simulink subsystem "Robot_Control_sub"  (R2026a)
settings: Solver=VariableStepAuto
undefined symbols (not defined in the file): Rebuilt_Hood_Servo_Pos_Max, Rebuilt_Hood_Servo_Pos_Min, TEST_Desired_Hood_Enable_OV, TEST_Desired_Hood_Pos_OV, TEST_Desired_Shooter_FF_DC_OV, TEST_Desired_Shooter_Speed_OV, TEST_Feeder_Motor_DC_OV, TEST_Intake_Arm_Motor_DC_OV, TEST_Intake_Roller_Motor_DC_OV, TEST_Output_Override_Flag, TEST_Transfer_Motor_DC_OV
libraries: Autonomous_lib x1, Disabled_lib x1, Controls_Components_lib x1, Teleop_lib x1, Test_lib x1
(part 1 of 2)
settings Model: Creator=USER  LastModifiedBy=ander

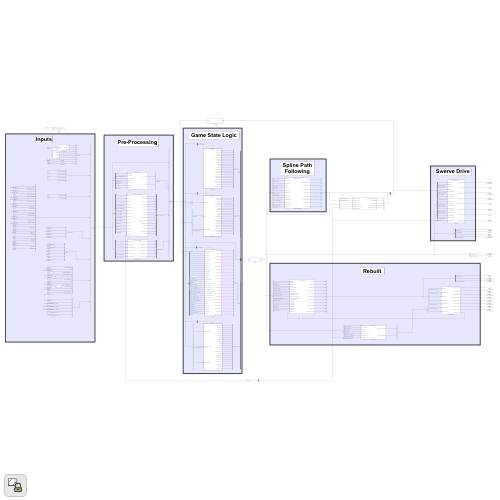
[thumbnail: Simulink's stored preview of the top-level diagram]
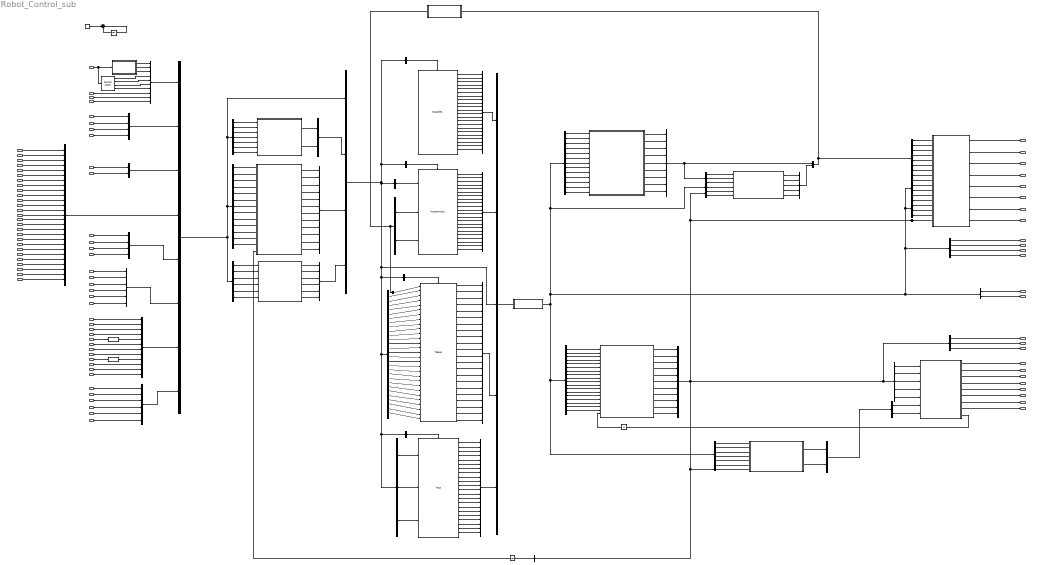
== system Robot_Control_sub ==
  note: Game State Logic
  note: Swerve Drive
  note: Inputs
  note: Pre-Processing
  note: Spline Path
      | Following
  note: Rebuilt
  GameState : Inport
  IsBlueAlliance : Inport  Port=2
  MatchTime : Inport  Port=3
  Xbox_Driver_Stick_Left_X : Inport  Port=4
  Xbox_Driver_Stick_Left_Y : Inport  Port=5
  Xbox_Driver_Bumper_Left : Inport  Port=6
  Xbox_Driver_Stick_Right_X : Inport  Port=7
  Xbox_Driver_Stick_Right_Y : Inport  Port=8
  Xbox_Driver_Bumper_Right : Inport  Port=9
  Xbox_Driver_Trigger_Right : Inport  Port=10
  Xbox_Driver_ButtonY : Inport  Port=11
  Xbox_Driver_ButtonX : Inport  Port=12
  Xbox_Driver_ButtonB : Inport  Port=13
  Xbox_Driver_ButtonA : Inport  Port=14
  Xbox_Driver_Trigger_Left : Inport  Port=15
  Gamepad_Stick_Left_X : Inport  Port=16
  Gamepad_Stick_Left_Y : Inport  Port=17
  Gamepad_Stick_Right_X : Inport  Port=18
  Gamepad_Stick_Right_Y : Inport  Port=19
  Gamepad_B1_A : Inport  Port=20
  Gamepad_B2_B : Inport  Port=21
  Gamepad_B3_X : Inport  Port=22
  Gamepad_B4_Y : Inport  Port=23
  Gamepad_LB : Inport  Port=24
  Gamepad_LT : Inport  Port=25
  Gamepad_RB : Inport  Port=26
  Gamepad_RT : Inport  Port=27
  Gamepad_Back : Inport  Port=28
  Gamepad_Start : Inport  Port=29
  Gamepad_POV : Inport  Port=30
  FL_Drive_Motor_Speed : Inport  Port=31
  FR_Drive_Motor_Speed : Inport  Port=32
  BL_Drive_Motor_Speed : Inport  Port=33
  BR_Drive_Motor_Speed : Inport  Port=34
  Gyro_Angle_Field_rad : Inport  Port=35
  Gyro_Angle_rad : Inport  Port=36
  FL_Steer_Module_Angle : Inport  Port=37
  FR_Steer_Module_Angle : Inport  Port=38
  BL_Steer_Module_Angle : Inport  Port=39
  BR_Steer_Module_Angle : Inport  Port=40
  Odom_Position_X : Inport  Port=41
  Odom_Position_Y : Inport  Port=42
  Odom_Delta_X : Inport  Port=43
  Odom_Delta_Y : Inport  Port=44
  Robot_Velocity_X : Inport  Port=45
  Robot_Velocity_Y : Inport  Port=46
  Vision_Current_Pipeline : Inport  Port=47
  Vision_RobotPoseFieldSpace_X : Inport  Port=48
  Vision_RobotPoseFieldSpace_Y : Inport  Port=49
  Vision_Num_Tags_Detected : Inport  Port=50
  Vision_c1_AprilTag_Valid : Inport  Port=51
  Vision_c1_AprilTag_X_m : Inport  Port=52
  Vision_c1_AprilTag_Y_m : Inport  Port=53
  Vision_c1_AprilTag_Yaw_deg : Inport  Port=54
  Vision_c1_Object_Valid : Inport  Port=55
  Vision_c1_Object_Area_pct : Inport  Port=56
  Vision_c1_Object_Hor_deg : Inport  Port=57
  Vision_c1_Object_Ver_deg : Inport  Port=58
  Measured_Transfer_Speed : Inport  Port=59
  Measured_Shooter_Speed_Left : Inport  Port=60
  Measured_Shooter_Speed_Center : Inport  Port=61
  Measured_Shooter_Speed_Right : Inport  Port=62
  IsBlueInactiveFirst : Inport  Port=63
  Measured_Intake_Arm_Angle : Inport  Port=64
  Measured_Intake_Roller_Speed : Inport  Port=65
  Autonomous : Autonomous_lib/Autonomous  SystemSampleTime=-1  VariantActivationTime=update diagram  EmptyChoice=off  PassThrough=off  PassThroughVariantControl=(default)  EmptyChoiceVariantControl=(default)  AllowFlexibleInterface=on  Latency=0  AutoFrameSizeCalculation=off
  Bus Creator : BusCreator  Inputs=10
  Bus Creator{1..2,4,12} (4 alike) : BusCreator  Inputs=22
  Bus Creator10 : BusCreator  Inputs=11
  Bus Creator11 : BusCreator  Inputs=8
  Bus Creator13 : BusCreator  Inputs=9
  Bus Creator{14,16,19..20} (4 alike) : BusCreator  Inputs=2
  Bus Creator15 : BusCreator  Inputs=5
  Bus Creator17 : BusCreator  Inputs=4
  Bus Creator18 : BusCreator  Inputs=12
  Bus Creator21 : BusCreator  Inputs=6
  Bus Creator24 : BusCreator  Inputs=12
  Bus Creator3 : BusCreator  Inputs=5
  Bus Creator5 : BusCreator  Inputs=27
  Bus Creator6 : BusCreator  Inputs=6
  Bus Creator7 : BusCreator  Inputs=4
  Bus Creator8 : BusCreator  Inputs=4
  Bus Creator9 : BusCreator  Inputs=6
  Bus Selector : BusSelector  OutputSignals=Desired_Gyro_Override.Steering_Abs_Cmd,SPF.Steering_Rel_Cmd_SPF,SPF.Translation_Speed_SPF,SPF.Translation_Angle_SPF,SPF.Is_Absolute_Translation_SPF,Desired_Gyro_Override.Is_Absolute_Steering,Desired_Gyro_Override.Gyro_Angle_Steering_rad,Desired_Gyro_Override.Gyro_Angle_Translation_rad
  Bus Selector1 : BusSelector  OutputSignals=PreProcessing.Inputs.Game_States.GameState,PreProcessing.Inputs.Game_States.IsBlueAlliance,PreProcessing.Inputs.Game_States.IsBlueInactiveFirst,PreProcessing.Inputs.Game_States.MatchTime,Button_Spinup_Enable,Button_Shoot_Enable,PreProcessing.Inputs.Human_Inputs_Raw.Gamepad_RT,PreProcessing.Inputs.Rebuilt_Specific.Measured_Transfer_Speed,PreProcessing.Inputs.Rebuilt_Specific.Measured_Shooter_Speed_Left,PreProcessing.Inputs.Rebuilt_Specific.Measured_Shooter_Speed_Center,PreProcessing.Inputs.Rebuilt_Specific.Measured_Shooter_Speed_Right,PreProcessing.Inputs.Gyro.Gyro_Angle_Field_rad,PreProcessing.Kalman_Filter.KF_Position_X,PreProcessing.Kalman_Filter.KF_Position_Y,PreProcessing.Inputs.Odometry.Robot_Velocity_X,PreProcessing.Inputs.Odometry.Robot_Velocity_Y,PreProcessing.Inputs.Human_Inputs_Raw.Gamepad_B2_B,PreProcessing.Inputs.Human_Inputs_Raw.Gamepad_Start
  Bus Selector10 : BusSelector  OutputSignals=Is_Absolute_Steering_SPF,Steering_Abs_Cmd_SPF,Gyro_Angle_SPF
  Bus Selector11 : BusSelector  OutputSignals=PreProcessing.Inputs.Gyro.Gyro_Angle_Field_rad
  Bus Selector12 : BusSelector  OutputSignals=Rebuilt_Intake_Arm_Motor_DC,RB_Intake_Roller_Motor_PID_DC
  Bus Selector13 : BusSelector  OutputSignals=Human_Inputs_Raw.Xbox_Driver_Stick_Left_X,Human_Inputs_Raw.Xbox_Driver_Stick_Left_Y,Human_Inputs_Raw.Xbox_Driver_Stick_Right_X,Human_Inputs_Raw.Xbox_Driver_Stick_Right_Y,Human_Inputs_Raw.Xbox_Driver_Trigger_Right,Human_Inputs_Raw.Xbox_Driver_ButtonY,Human_Inputs_Raw.Xbox_Driver_ButtonX,Human_Inputs_Raw.Xbox_Driver_ButtonB,Human_Inputs_Raw.Xbox_Driver_ButtonA,Human_Inputs_Raw.Gamepad_B3_X,Human_Inputs_Raw.Gamepad_B4_Y,Human_Inputs_Raw.Gamepad_B2_B,Gyro.Gyro_Angle_rad
  Bus Selector14 : BusSelector  OutputSignals=Intake_Arm_Move_In,Intake_Arm_Move_Out,Intake_Arm_Cycle,Intake_Roller_On,PreProcessing.Inputs.Rebuilt_Specific.Measured_Intake_Arm_Angle,PreProcessing.Inputs.Rebuilt_Specific.Measured_Intake_Roller_Speed
  Bus Selector15 : BusSelector  OutputSignals=Spline_Index,Robot_Reached_Destination
  Bus Selector16 : BusSelector  OutputSignals=Human_Inputs_Processed.Button_Enable_Wheels,Human_Inputs_Processed.Button_Reset_Wheel_Offsets,Human_Inputs_Processed.Button_Disable_Wheels
  Bus Selector17 : BusSelector  OutputSignals=Field_Angle_Override_Enable
  Bus Selector18 : BusSelector  OutputSignals=Enable_Wheels,Reset_Wheel_Offsets,Disable_Wheels,Swerve_Motors_Disabled
  Bus Selector19 : BusSelector  OutputSignals=Desired_Pipeline,Auto_Initial_Gyro_Angle
  Bus Selector2 : BusSelector  OutputSignals=Inputs.Game_States.Game_State_Teleop
  Bus Selector20 : BusSelector  OutputSignals=Vision_Estimates.Vision_c1_AprilTag_X_m,Vision_Estimates.Vision_c1_AprilTag_Y_m,Vision_Estimates.Vision_c1_AprilTag_Yaw_deg,Vision_Estimates.Vision_c1_Object_Area_pct,Vision_Estimates.Vision_c1_Object_Hor_deg,Vision_Estimates.Vision_c1_Object_Ver_deg
  Bus Selector22 : BusSelector  OutputSignals=Shooter_Active
  Bus Selector23 : BusSelector  OutputSignals=Aim_Active
  Bus Selector24 : BusSelector  OutputSignals=Shooter_Motor_Gain_Kp,Shooter_Motor_Gain_Ki,Shooter_Motor_Gain_Change
  Bus Selector25 : BusSelector  OutputSignals=RB_Transfer_Motor_PID_DC
  Bus Selector3 : BusSelector  OutputSignals=Vision_Estimates.Vision_RobotPoseFieldSpace_X,Vision_Estimates.Vision_RobotPoseFieldSpace_Y,Vision_Estimates.Vision_Num_Tags_Detected,Odometry.Odom_Position_X,Odometry.Odom_Position_Y,Odometry.Odom_Delta_X,Odometry.Odom_Delta_Y
  Bus Selector4 : BusSelector  OutputSignals=Inputs.Game_States.Game_State_Auto
  Bus Selector41 : BusSelector  OutputSignals=Human_Inputs_Processed.Drive_Joystick_X,Human_Inputs_Processed.Drive_Joystick_Y,Human_Inputs_Processed.Steer_Joystick_X,Human_Inputs_Processed.Steer_Joystick_Y,Human_Inputs_Processed.Drive_Speed_Boost,Human_Inputs_Processed.Face_Toward_Driver,Human_Inputs_Processed.Face_Right_Driver,Human_Inputs_Processed.Face_Left_Driver,Human_Inputs_Processed.Face_Away_Driver,Inputs.Gyro.Gyro_Angle_rad,Inputs.Game_States.Prev_Active_GameState,Inputs.Game_States.IsBlueAlliance,Inputs.Vision_Estimates.Vision_Current_Pipeline,Inputs.Vision_Estimates.Vision_c1_AprilTag_Valid,Vision_Corrected.Vision_c1_AprilTag_Corr_X_inch,Vision_Corrected.Vision_c1_AprilTag_Corr_Y_inch,Vision_Corrected.Vision_c1_AprilTag_Corr_Yaw_deg,Inputs.Vision_Estimates.Vision_c1_Object_Valid,Vision_Corrected.Vision_c1_Object_Corr_X_inch,Vision_Corrected.Vision_c1_Object_Corr_Y_inch,Vision_Corrected.Vision_c1_Object_Corr_Yaw_deg,Inputs.Human_Inputs_Raw.Gamepad_LB,Inputs.Human_Inputs_Raw.Gamepad_RB,Inputs.Human_Inputs_Raw.Gamepad_B1_A,Inputs.Human_Inputs_Raw.Gamepad_B4_Y,Inputs.Human_Inputs_Raw.Gamepad_B3_X,Inputs.Human_Inputs_Raw.Xbox_Driver_Trigger_Left,Inputs.Human_Inputs_Raw.Gamepad_LT
  Bus Selector5 : BusSelector  OutputSignals=Aim_Active,RB_Desired_Shoot_Gyro_Ang
  Bus Selector50 : BusSelector  OutputSignals=PreProcessing.Inputs.Drive_Motor_Speeds.FL_Drive_Motor_Speed,PreProcessing.Inputs.Drive_Motor_Speeds.FR_Drive_Motor_Speed,PreProcessing.Inputs.Drive_Motor_Speeds.BL_Drive_Motor_Speed,PreProcessing.Inputs.Drive_Motor_Speeds.BR_Drive_Motor_Speed
  Bus Selector52 : BusSelector  OutputSignals=PreProcessing.Inputs.Steer_Module_Angles.FL_Steer_Module_Angle,PreProcessing.Inputs.Steer_Module_Angles.FR_Steer_Module_Angle,PreProcessing.Inputs.Steer_Module_Angles.BL_Steer_Module_Angle,PreProcessing.Inputs.Steer_Module_Angles.BR_Steer_Module_Angle
  Bus Selector59 : BusSelector  OutputSignals=Inputs.Game_States.IsBlueAlliance
  Bus Selector6 : BusSelector  OutputSignals=Inputs.Game_States.Game_State_Disabled
  Bus Selector7 : BusSelector  OutputSignals=RB_Transfer_Motor_PID_DC,RB_Feeder_Motor_PID_DC,RB_Desired_Hood_Pos_Shoot,RB_Desired_Shooter_Speed,Desired_Shooter_FF_DC
  Bus Selector8 : BusSelector  OutputSignals=Inputs.Game_States.Game_State_Test
  Bus Selector9 : BusSelector  OutputSignals=Spline_Enable,Spline_Ref_Poses,Spline_Num_Poses,PreProcessing.Kalman_Filter.KF_Position_X,PreProcessing.Kalman_Filter.KF_Position_Y,Steering_Abs_Cmd,Steering_Rel_Cmd,Translation_Speed,Translation_Angle,Is_Absolute_Translation,Is_Absolute_Steering,PreProcessing.Inputs.Gyro.Gyro_Angle_Field_rad,PreProcessing.Inputs.Gyro.Gyro_Angle_rad
  Constant2 : Constant
  Data Type Conversion : DataTypeConversion  OutDataTypeStr=boolean  SaturateOnIntegerOverflow=off  RndMeth=Floor
  Data Type Conversion1 : DataTypeConversion  OutDataTypeStr=boolean  SaturateOnIntegerOverflow=off  RndMeth=Floor
  Desired Gyro Override for Shooting : Subsystem
  Disabled : Disabled_lib/Disabled  SystemSampleTime=-1  VariantActivationTime=update diagram  EmptyChoice=off  PassThrough=off  PassThroughVariantControl=(default)  EmptyChoiceVariantControl=(default)  AllowFlexibleInterface=on  Latency=0  AutoFrameSizeCalculation=off
  Human_Input_Pre_Processing : Subsystem  ReferencedSubsystem=Human_Input_Pre_Processing_sub
  Intake Controls : Subsystem  ReferencedSubsystem=Intake_Controls_sub
  Internal Feedback : Subsystem
  Kalman_Filter : Subsystem  ReferencedSubsystem=Kalman_Filter_sub
  Merge : Subsystem
  Output Overrides : Subsystem
  Previous GameState : Subsystem
  Shooter Controls : Subsystem  ReferencedSubsystem=Shooter_Controls_sub
  Spline_Path_Following : Subsystem  ReferencedSubsystem=Spline_Path_Following_sub
  Sum : Sum  Inputs=|++
  Swerve_Drive : Subsystem  ReferencedSubsystem=Swerve_Drive_sub
  Switch Case : SwitchCase  CaseConditions={0,1,2}
  Teleop : Teleop_lib/Teleop  SystemSampleTime=-1  VariantActivationTime=update diagram  EmptyChoice=off  PassThrough=off  PassThroughVariantControl=(default)  EmptyChoiceVariantControl=(default)  AllowFlexibleInterface=on  Latency=0  AutoFrameSizeCalculation=off
  Test : Test_lib/Test  SystemSampleTime=-1  VariantActivationTime=update diagram  EmptyChoice=off  PassThrough=off  PassThroughVariantControl=(default)  EmptyChoiceVariantControl=(default)  AllowFlexibleInterface=on  Latency=0  AutoFrameSizeCalculation=off
  Unit Delay : UnitDelay  SampleTime=-1
  Unit Delay1 : UnitDelay  SampleTime=-1
  Unit Delay2 : UnitDelay  SampleTime=-1
  Vision_Corrections : Subsystem  ReferencedSubsystem=Vision_Corrections_sub
  FL_Steering_Motor_DC : Outport
  FL_Drive_Motor_DC : Outport  Port=2
  FR_Steering_Motor_DC : Outport  Port=3
  FR_Drive_Motor_DC : Outport  Port=4
  BL_Steering_Motor_DC : Outport  Port=5
  BL_Drive_Motor_DC : Outport  Port=6
  BR_Steering_Motor_DC : Outport  Port=7
  BR_Drive_Motor_DC : Outport  Port=8
  Enable_Wheels : Outport  Port=9
  Reset_Wheel_Offsets : Outport  Port=10
  Disable_Wheels : Outport  Port=11
  Swerve_Motors_Disabled : Outport  Port=12
  Vision_Desired_Pipeline : Outport  Port=13
  Transfer_Motor_DC : Outport  Port=14
  Feeder_Motor_DC : Outport  Port=15
  Desired_Shooter_Speed : Outport  Port=16
  Desired_Shooter_FF_DC : Outport  Port=17
  Desired_Hood_Enable : Outport  Port=18
  Desired_Hood_Pos : Outport  Port=19
  Intake_Arm_Motor_DC : Outport  Port=20
  Intake_Roller_Motor_DC : Outport  Port=21
  Auto_Initial_Gyro_Angle : Outport  Port=22
  Shooter_Motor_Gain_Kp : Outport  Port=23
  Shooter_Motor_Gain_Ki : Outport  Port=24
  Shooter_Motor_Gain_Change : Outport  Port=25
  wires:
  Bus Creator4/1 -> Bus Creator3/1  "Disabled"
  Bus Creator1/1 -> Bus Creator3/2  "Autonomous"
  Bus Creator2/1 -> Bus Creator3/4  "Teleop"
  Switch Case/1 -> Bus Creator/4  "Game_State_Disabled"
  Switch Case/2 -> Bus Creator/5  "Game_State_Auto"
  Switch Case/3 -> Bus Creator/6  "Game_State_Teleop"
  GameState/1 -> Previous GameState/1(GameState_in), Switch Case/1  "GameState"
  Bus Creator12/1 -> Bus Creator3/5  "Test"
  Switch Case/4 -> Bus Creator/7  "Game_State_Test"
  FL_Drive_Motor_Speed/1 -> Bus Creator7/1  "FL_Drive_Motor_Speed"
  FR_Drive_Motor_Speed/1 -> Bus Creator7/2  "FR_Drive_Motor_Speed"
  BL_Drive_Motor_Speed/1 -> Bus Creator7/3  "BL_Drive_Motor_Speed"
  BR_Drive_Motor_Speed/1 -> Bus Creator7/4  "BR_Drive_Motor_Speed"
  Bus Creator/1 -> Bus Creator11/1  "Game_States"
  Bus Selector2/1 -> Teleop/Action  "<Game_State_Teleop>"
  Bus Selector4/1 -> Autonomous/Action  "<Game_State_Auto>"
  Bus Selector6/1 -> Disabled/Action  "<Game_State_Disabled>"
  Bus Selector8/1 -> Test/Action  "<Game_State_Test>"
  Bus Selector50/4 -> Swerve_Drive/12  "<BR_Drive_Motor_Speed>"
  Bus Selector50/3 -> Swerve_Drive/11  "<BL_Drive_Motor_Speed>"
  Bus Selector50/2 -> Swerve_Drive/10  "<FR_Drive_Motor_Speed>"
  Bus Selector50/1 -> Swerve_Drive/9  "<FL_Drive_Motor_Speed>"
  Swerve_Drive/1 -> FL_Steering_Motor_DC/1
  Swerve_Drive/2 -> FL_Drive_Motor_DC/1
  Swerve_Drive/3 -> FR_Steering_Motor_DC/1
  Swerve_Drive/4 -> FR_Drive_Motor_DC/1
  Swerve_Drive/5 -> BL_Steering_Motor_DC/1
  Swerve_Drive/6 -> BL_Drive_Motor_DC/1
  Swerve_Drive/7 -> BR_Steering_Motor_DC/1
  Swerve_Drive/8 -> BR_Drive_Motor_DC/1
  Xbox_Driver_Trigger_Right/1 -> Bus Creator5/8  "Xbox_Driver_Trigger_Right"
  Gyro_Angle_Field_rad/1 -> Bus Creator14/1  "Gyro_Angle_Field_rad"
  Gyro_Angle_rad/1 -> Bus Creator14/2  "Gyro_Angle_rad"
  Bus Creator11/1 -> Bus Selector20/1, Bus Selector13/1, Bus Selector3/1, Bus Creator17/1  "Inputs"
  Bus Selector52/1 -> Swerve_Drive/13  "<FL_Steer_Module_Angle>"
  Bus Selector52/2 -> Swerve_Drive/14  "<FR_Steer_Module_Angle>"
  Bus Selector52/3 -> Swerve_Drive/15  "<BL_Steer_Module_Angle>"
  Bus Selector52/4 -> Swerve_Drive/16  "<BR_Steer_Module_Angle>"
  Merge/1(Bus_Out) -> Bus Selector11/1, Bus Selector9/1, Bus Selector19/1, Bus Selector18/1, Bus Selector52/1, Bus Selector50/1, Bus Selector1/1, Bus Selector14/1
  Bus Creator3/1 -> Merge/1(Bus_In)
  Bus Selector9/1 -> Spline_Path_Following/1  "<Spline_Enable>"
  Bus Selector9/2 -> Spline_Path_Following/2  "<Spline_Ref_Poses>"
  Bus Selector9/3 -> Spline_Path_Following/3  "<Spline_Num_Poses>"
  Bus Selector9/7 -> Spline_Path_Following/7  "<Steering_Rel_Cmd>"
  Bus Selector9/8 -> Spline_Path_Following/8  "<Translation_Speed>"
  Bus Selector9/9 -> Spline_Path_Following/9  "<Translation_Angle>"
  Bus Selector9/10 -> Spline_Path_Following/10  "<Is_Absolute_Translation>"
  Bus Selector9/11 -> Spline_Path_Following/11  "<Is_Absolute_Steering>"
  Spline_Path_Following/3 -> Bus Creator13/3
  Spline_Path_Following/4 -> Bus Creator13/4
  Spline_Path_Following/5 -> Bus Creator13/5
  Spline_Path_Following/6 -> Bus Creator13/6
  Spline_Path_Following/7 -> Bus Creator13/7
  Spline_Path_Following/8 -> Bus Creator13/8
  Bus Creator13/1 -> Bus Creator16/1, Bus Selector10/1  "SPF"
  Bus Selector/5 -> Swerve_Drive/5  "<Is_Absolute_Translation_SPF>"
  Bus Selector/4 -> Swerve_Drive/4  "<Translation_Angle_SPF>"
  Bus Selector/6 -> Swerve_Drive/6  "<Is_Absolute_Steering>"
  Bus Selector/3 -> Swerve_Drive/3  "<Translation_Speed_SPF>"
  Bus Selector/2 -> Swerve_Drive/2  "<Steering_Rel_Cmd_SPF>"
  Bus Selector/1 -> Swerve_Drive/1  "<Steering_Abs_Cmd>"
  Spline_Path_Following/2 -> Bus Creator13/2
  Vision_RobotPoseFieldSpace_X/1 -> Bus Creator18/2  "Vision_RobotPoseFieldSpace_X"
  Vision_RobotPoseFieldSpace_Y/1 -> Bus Creator18/3  "Vision_RobotPoseFieldSpace_Y"
  Vision_Num_Tags_Detected/1 -> Bus Creator18/4  "Vision_Num_Tags_Detected"
  Bus Selector3/3 -> Kalman_Filter/3  "<Vision_Num_Tags_Detected>"
  Bus Selector3/2 -> Kalman_Filter/2  "<Vision_RobotPoseFieldSpace_Y>"
  Bus Selector3/1 -> Kalman_Filter/1  "<Vision_RobotPoseFieldSpace_X>"
  Kalman_Filter/1 -> Bus Creator19/1
  Kalman_Filter/2 -> Bus Creator19/2
  Bus Selector9/4 -> Spline_Path_Following/4  "<KF_Position_X>"
  Bus Selector9/5 -> Spline_Path_Following/5  "<KF_Position_Y>"
  Bus Creator19/1 -> Bus Creator17/2  "Kalman_Filter"
  Xbox_Driver_ButtonB/1 -> Bus Creator5/11  "Xbox_Driver_ButtonB"
  Xbox_Driver_ButtonX/1 -> Bus Creator5/10  "Xbox_Driver_ButtonX"
  Xbox_Driver_ButtonY/1 -> Bus Creator5/9  "Xbox_Driver_ButtonY"
  Bus Selector13/3 -> Human_Input_Pre_Processing/3  "<Xbox_Driver_Stick_Right_X>"
  Bus Selector13/4 -> Human_Input_Pre_Processing/4  "<Xbox_Driver_Stick_Right_Y>"
  Bus Selector13/1 -> Human_Input_Pre_Processing/1  "<Xbox_Driver_Stick_Left_X>"
  Bus Selector13/2 -> Human_Input_Pre_Processing/2  "<Xbox_Driver_Stick_Left_Y>"
  Bus Selector13/5 -> Human_Input_Pre_Processing/5  "<Xbox_Driver_Trigger_Right>"
  Xbox_Driver_Stick_Left_Y/1 -> Bus Creator5/2  "Xbox_Driver_Stick_Left_Y"
  Xbox_Driver_Stick_Left_X/1 -> Bus Creator5/1  "Xbox_Driver_Stick_Left_X"
  Xbox_Driver_Bumper_Left/1 -> Bus Creator5/5  "Xbox_Driver_Bumper_Left"
  Xbox_Driver_Stick_Right_X/1 -> Bus Creator5/3  "Xbox_Driver_Stick_Right_X"
  Xbox_Driver_Stick_Right_Y/1 -> Bus Creator5/4  "Xbox_Driver_Stick_Right_Y"
  Xbox_Driver_Bumper_Right/1 -> Bus Creator5/6  "Xbox_Driver_Bumper_Right"
  Bus Creator24/1 -> Bus Creator17/3  "Human_Inputs_Processed"
  Bus Creator17/1 -> Bus Selector4/1, Bus Selector6/1, Bus Creator3/3, Bus Selector2/1, Bus Selector41/1, Bus Selector8/1, Bus Selector16/1, Bus Selector59/1  "PreProcessing"
  Bus Creator18/1 -> Bus Creator11/7  "Vision_Estimates"
  Vision_c1_AprilTag_X_m/1 -> Bus Creator18/6  "Vision_c1_AprilTag_X_m"
  Vision_c1_AprilTag_Y_m/1 -> Bus Creator18/7  "Vision_c1_AprilTag_Y_m"
  Previous GameState/1(GameState) -> Bus Creator/1
  Previous GameState/3(Prev_Active_GameState) -> Bus Creator/3
  IsBlueAlliance/1 -> Bus Creator/8  "IsBlueAlliance"
  Bus Selector9/12 -> Spline_Path_Following/12  "<Gyro_Angle_Field_rad>"
  Bus Selector9/13 -> Spline_Path_Following/13  "<Gyro_Angle_rad>"
  Spline_Path_Following/9 -> Bus Creator13/9
  Bus Selector59/1 -> Autonomous/1  "<IsBlueAlliance>"
  Bus Selector18/2 -> Reset_Wheel_Offsets/1  "<Reset_Wheel_Offsets>"
  Bus Selector18/3 -> Disable_Wheels/1  "<Disable_Wheels>"
  Bus Selector18/4 -> Swerve_Motors_Disabled/1  "<Swerve_Motors_Disabled>"
  Bus Selector18/1 -> Enable_Wheels/1  "<Enable_Wheels>"
  Bus Selector16/1 -> Test/1  "<Button_Enable_Wheels>"
  Bus Selector16/2 -> Test/2  "<Button_Reset_Wheel_Offsets>"
  Bus Selector16/3 -> Test/3  "<Button_Disable_Wheels>"
  Xbox_Driver_ButtonA/1 -> Bus Creator5/12  "Xbox_Driver_ButtonA"
  Xbox_Driver_Trigger_Left/1 -> Bus Creator5/7  "Xbox_Driver_Trigger_Left"
  Gamepad_Stick_Left_X/1 -> Bus Creator5/13  "Gamepad_Stick_Left_X"
  Gamepad_Stick_Left_Y/1 -> Bus Creator5/14  "Gamepad_Stick_Left_Y"
  Gamepad_Stick_Right_X/1 -> Bus Creator5/15  "Gamepad_Stick_Right_X"
  Gamepad_Stick_Right_Y/1 -> Bus Creator5/16  "Gamepad_Stick_Right_Y"
  Gamepad_B1_A/1 -> Bus Creator5/17  "Gamepad_B1_A"
  Gamepad_B2_B/1 -> Bus Creator5/18  "Gamepad_B2_B"
  Gamepad_B3_X/1 -> Bus Creator5/19  "Gamepad_B3_X"
  Gamepad_B4_Y/1 -> Bus Creator5/20  "Gamepad_B4_Y"
  Gamepad_LB/1 -> Bus Creator5/21  "Gamepad_LB"
  Gamepad_LT/1 -> Bus Creator5/22  "Gamepad_LT"
  Gamepad_RB/1 -> Bus Creator5/23  "Gamepad_RB"
  Gamepad_RT/1 -> Bus Creator5/24  "Gamepad_RT"
  Gamepad_Back/1 -> Bus Creator5/25  "Gamepad_Back"
  Gamepad_Start/1 -> Bus Creator5/26  "Gamepad_Start"
  Bus Creator5/1 -> Bus Creator11/4  "Human_Inputs_Raw"
  Gamepad_POV/1 -> Bus Creator5/27  "Gamepad_POV"
  Vision_Corrections/1 -> Bus Creator21/1
  Vision_Corrections/2 -> Bus Creator21/2
  Vision_Corrections/3 -> Bus Creator21/3
  Bus Creator21/1 -> Bus Creator17/4  "Vision_Corrected"
  Previous GameState/2(Prev_GameState) -> Bus Creator/2
  MatchTime/1 -> Bus Creator/9  "MatchTime"
  Odom_Position_X/1 -> Bus Creator9/1  "Odom_Position_X"
  Odom_Position_Y/1 -> Bus Creator9/2  "Odom_Position_Y"
  Odom_Delta_X/1 -> Bus Creator9/3  "Odom_Delta_X"
  Odom_Delta_Y/1 -> Bus Creator9/4  "Odom_Delta_Y"
  Bus Creator9/1 -> Bus Creator11/6  "Odometry"
  BR_Steer_Module_Angle/1 -> Bus Creator8/4  "BR_Steer_Module_Angle"
  BL_Steer_Module_Angle/1 -> Bus Creator8/3  "BL_Steer_Module_Angle"
  FR_Steer_Module_Angle/1 -> Bus Creator8/2  "FR_Steer_Module_Angle"
  FL_Steer_Module_Angle/1 -> Bus Creator8/1  "FL_Steer_Module_Angle"
  Bus Creator7/1 -> Bus Creator11/2  "Drive_Motor_Speeds"
  Bus Creator14/1 -> Bus Creator11/3  "Gyro"
  Constant2/1 -> Sum/1
  Unit Delay1/1 -> Sum/2
  Sum/1 -> Unit Delay1/1  "loop_counter_robot_control"
  Vision_c1_AprilTag_Yaw_deg/1 -> Bus Creator18/8  "Vision_c1_AprilTag_Yaw_deg"
  Teleop/1 -> Bus Creator2/1
  Teleop/2 -> Bus Creator2/2
  Teleop/3 -> Bus Creator2/3
  Teleop/4 -> Bus Creator2/4
  Teleop/5 -> Bus Creator2/5
  Teleop/6 -> Bus Creator2/6
  Teleop/7 -> Bus Creator2/7
  Test/1 -> Bus Creator12/1
  Test/2 -> Bus Creator12/2
  Test/3 -> Bus Creator12/3
  Test/4 -> Bus Creator12/4
  Test/5 -> Bus Creator12/5
  Test/6 -> Bus Creator12/6
  Test/7 -> Bus Creator12/7
  Test/8 -> Bus Creator12/8
  Test/9 -> Bus Creator12/9
  Test/10 -> Bus Creator12/10
  Test/11 -> Bus Creator12/11
  Test/12 -> Bus Creator12/12
  Test/13 -> Bus Creator12/13
  Test/14 -> Bus Creator12/14
  Disabled/1 -> Bus Creator4/1
  Disabled/2 -> Bus Creator4/2
  Disabled/3 -> Bus Creator4/3
  Disabled/4 -> Bus Creator4/4
  Disabled/5 -> Bus Creator4/5
  Disabled/6 -> Bus Creator4/6
  Disabled/7 -> Bus Creator4/7
  Disabled/8 -> Bus Creator4/8
  Disabled/9 -> Bus Creator4/9
  Disabled/10 -> Bus Creator4/10
  Disabled/11 -> Bus Creator4/11
  Disabled/12 -> Bus Creator4/12
  Disabled/13 -> Bus Creator4/13
  Disabled/14 -> Bus Creator4/14
  Autonomous/1 -> Bus Creator1/1
  Autonomous/2 -> Bus Creator1/2
  Autonomous/3 -> Bus Creator1/3
  Autonomous/4 -> Bus Creator1/4
  Autonomous/5 -> Bus Creator1/5
  Autonomous/6 -> Bus Creator1/6
  Autonomous/7 -> Bus Creator1/7
  Autonomous/8 -> Bus Creator1/8
  Autonomous/9 -> Bus Creator1/9
  Autonomous/10 -> Bus Creator1/10
  Autonomous/11 -> Bus Creator1/11
  Autonomous/12 -> Bus Creator1/12
  Autonomous/13 -> Bus Creator1/13
  Autonomous/14 -> Bus Creator1/14
  Bus Creator8/1 -> Bus Creator11/5  "Steer_Module_Angles"
  Vision_Current_Pipeline/1 -> Bus Creator18/1  "Vision_Current_Pipeline"
  Bus Selector20/1 -> Vision_Corrections/1  "<Vision_c1_AprilTag_X_m>"
  Vision_c1_Object_Area_pct/1 -> Bus Creator18/10  "Vision_c1_Object_Area_pct"
  Vision_c1_Object_Hor_deg/1 -> Bus Creator18/11  "Vision_c1_Object_Hor_deg"
  Vision_c1_Object_Ver_deg/1 -> Bus Creator18/12  "Vision_c1_Object_Ver_deg"
  Vision_Corrections/4 -> Bus Creator21/4
  Vision_Corrections/5 -> Bus Creator21/5
  Vision_Corrections/6 -> Bus Creator21/6
  Vision_c1_AprilTag_Valid/1 -> Data Type Conversion1/1
  Vision_c1_Object_Valid/1 -> Data Type Conversion/1
  Bus Selector3/4 -> Kalman_Filter/4  "<Odom_Position_X>"
  Bus Selector3/5 -> Kalman_Filter/5  "<Odom_Position_Y>"
  Bus Selector3/6 -> Kalman_Filter/6  "<Odom_Delta_X>"
  Bus Selector3/7 -> Kalman_Filter/7  "<Odom_Delta_Y>"
  Data Type Conversion/1 -> Bus Creator18/9  "Vision_c1_Object_Valid"
  Data Type Conversion1/1 -> Bus Creator18/5  "Vision_c1_AprilTag_Valid"
  Bus Selector1/1 -> Shooter Controls/1  "<GameState>"
  Bus Selector1/2 -> Shooter Controls/2  "<IsBlueAlliance>"
  Bus Selector1/4 -> Shooter Controls/4  "<MatchTime>"
  Bus Selector1/5 -> Shooter Controls/5  "<Button_Spinup_Enable>"
  Bus Selector1/6 -> Shooter Controls/6  "<Button_Shoot_Enable>"
  Bus Selector1/3 -> Shooter Controls/3  "<IsBlueInactiveFirst>"
  Bus Creator6/1 -> Bus Creator11/8  "Rebuilt_Specific"
  Measured_Transfer_Speed/1 -> Bus Creator6/1  "Measured_Transfer_Speed"
  Measured_Shooter_Speed_Left/1 -> Bus Creator6/2  "Measured_Shooter_Speed_Left"
  Measured_Shooter_Speed_Center/1 -> Bus Creator6/3  "Measured_Shooter_Speed_Center"
  Measured_Shooter_Speed_Right/1 -> Bus Creator6/4  "Measured_Shooter_Speed_Right"
  Bus Selector1/8 -> Shooter Controls/8  "<Measured_Transfer_Speed>"
  Bus Selector1/9 -> Shooter Controls/9  "<Measured_Shooter_Speed_Left>"
  Bus Selector1/10 -> Shooter Controls/10  "<Measured_Shooter_Speed_Center>"
  Bus Selector1/11 -> Shooter Controls/11  "<Measured_Shooter_Speed_Right>"
  Bus Selector1/12 -> Shooter Controls/12  "<Gyro_Angle_Field_rad>"
  Bus Selector1/13 -> Shooter Controls/13  "<KF_Position_X>"
  Bus Selector1/14 -> Shooter Controls/14  "<KF_Position_Y>"
  Robot_Velocity_X/1 -> Bus Creator9/5  "Robot_Velocity_X"
  Robot_Velocity_Y/1 -> Bus Creator9/6  "Robot_Velocity_Y"
  Bus Selector1/15 -> Shooter Controls/15  "<Robot_Velocity_X>"
  Bus Selector1/16 -> Shooter Controls/16  "<Robot_Velocity_Y>"
  Shooter Controls/2 -> Bus Creator10/2
  Shooter Controls/3 -> Bus Creator10/3
  Shooter Controls/4 -> Bus Creator10/4
  Shooter Controls/5 -> Bus Creator10/5
  Shooter Controls/6 -> Bus Creator10/6
  Bus Creator10/1 -> Bus Selector7/1, Bus Selector24/1, Bus Selector23/1, Bus Selector5/1, Bus Selector25/1, Bus Selector22/1
  Bus Selector7/1 -> Output Overrides/1(Transfer_Motor_DC)  "<RB_Transfer_Motor_PID_DC>"
  Bus Selector7/2 -> Output Overrides/2(Feeder_Motor_DC)  "<RB_Feeder_Motor_PID_DC>"
  Bus Selector7/3 -> Output Overrides/3(Desired_Hood_Pos)  "<RB_Desired_Hood_Pos_Shoot>"
  Output Overrides/1(Transfer_Motor_DC_out) -> Transfer_Motor_DC/1
  Output Overrides/2(Feeder_Motor_DC_out) -> Feeder_Motor_DC/1
  Output Overrides/3(Desired_Shooter_Speed_out) -> Desired_Shooter_Speed/1
  Output Overrides/4(Desired_Shooter_FF_DC_out) -> Desired_Shooter_FF_DC/1
  Output Overrides/6(Desired_Hood_Pos_out) -> Desired_Hood_Pos/1
  Output Overrides/5(Desired_Hood_Enable_out) -> Desired_Hood_Enable/1
  IsBlueInactiveFirst/1 -> Bus Creator/10  "IsBlueInactiveFirst"
  Output Overrides/9(Estimated_Hood_Pos) -> Unit Delay/1
  Unit Delay/1 -> Shooter Controls/19
  Bus Selector9/6 -> Spline_Path_Following/6  "<Steering_Abs_Cmd>"
  Bus Selector10/1 -> Desired Gyro Override for Shooting/1(Is_Absolute_Steering_SPF)  "<Is_Absolute_Steering_SPF>"
  Bus Selector10/2 -> Desired Gyro Override for Shooting/2(Steering_Abs_Cmd_SPF)  "<Steering_Abs_Cmd_SPF>"
  Bus Selector10/3 -> Desired Gyro Override for Shooting/3(Gyro_Angle_SPF)  "<Gyro_Angle_SPF>"
  Bus Selector5/2 -> Desired Gyro Override for Shooting/6(Field_Angle_Override_rad)  "<RB_Desired_Shoot_Gyro_Ang>"
  Shooter Controls/1 -> Bus Creator10/1
  Bus Selector5/1 -> Desired Gyro Override for Shooting/5(Field_Angle_Override_Enable)  "<Aim_Active>"
  Bus Selector11/1 -> Desired Gyro Override for Shooting/4(Gyro_Angle_Field_rad)  "<Gyro_Angle_Field_rad>"
  Desired Gyro Override for Shooting/3(Steering_Abs_Cmd) -> Bus Creator15/3
  Desired Gyro Override for Shooting/2(Is_Absolute_Steering) -> Bus Creator15/2
  Bus Creator15/1 -> Bus Creator16/2  "Desired_Gyro_Override"
  Bus Creator16/1 -> Bus Selector/1, Internal Feedback/1(Bus_In)
  Desired Gyro Override for Shooting/4(Gyro_Angle_Steering_rad) -> Bus Creator15/4
  Desired Gyro Override for Shooting/5(Gyro_Angle_Translation_rad) -> Bus Creator15/5
  Bus Selector/7 -> Swerve_Drive/7  "<Gyro_Angle_Steering_rad>"
  Bus Selector/8 -> Swerve_Drive/8  "<Gyro_Angle_Translation_rad>"
  Intake Controls/1 -> Bus Creator20/1
  Intake Controls/2 -> Bus Creator20/2
  Bus Creator20/1 -> Bus Selector12/1
  Bus Selector12/1 -> Output Overrides/6(Intake_Arm_Motor_DC)  "<Rebuilt_Intake_Arm_Motor_DC>"
  Bus Selector12/2 -> Output Overrides/7(Intake_Roller_Motor_DC)  "<RB_Intake_Roller_Motor_PID_DC>"
  Output Overrides/7(Intake_Arm_Motor_DC_out) -> Intake_Arm_Motor_DC/1
  Output Overrides/8(Intake_Roller_Motor_DC_out) -> Intake_Roller_Motor_DC/1
  Measured_Intake_Arm_Angle/1 -> Bus Creator6/5  "Measured_Intake_Arm_Angle"
  Measured_Intake_Roller_Speed/1 -> Bus Creator6/6  "Measured_Intake_Roller_Speed"
  Bus Selector14/5 -> Intake Controls/5  "<Measured_Intake_Arm_Angle>"
  Bus Selector14/6 -> Intake Controls/6  "<Measured_Intake_Roller_Speed>"
  Bus Selector14/1 -> Intake Controls/1  "<Intake_Arm_Move_In>"
  Bus Selector14/2 -> Intake Controls/2  "<Intake_Arm_Move_Out>"
  Bus Selector14/3 -> Intake Controls/3  "<Intake_Arm_Cycle>"
  Bus Selector14/4 -> Intake Controls/4  "<Intake_Roller_On>"
  Desired Gyro Override for Shooting/1(Field_Angle_Override_Enable_out) -> Bus Creator15/1
  Bus Selector41/1 -> Teleop/2  "<Drive_Joystick_X>"
  Bus Selector41/2 -> Teleop/3  "<Drive_Joystick_Y>"
  Spline_Path_Following/1 -> Bus Creator13/1
  Internal Feedback/1(Bus_Out) -> Bus Selector15/1, Bus Selector17/1
  Bus Selector15/1 -> Autonomous/2  "<Spline_Index>"
  Bus Selector15/2 -> Autonomous/3  "<Robot_Reached_Destination>"
  Bus Selector17/1 -> Teleop/1  "<Field_Angle_Override_Enable>"
  Bus Selector19/1 -> Vision_Desired_Pipeline/1  "<Desired_Pipeline>"
  Bus Selector19/2 -> Auto_Initial_Gyro_Angle/1  "<Auto_Initial_Gyro_Angle>"
  Bus Selector20/2 -> Vision_Corrections/2  "<Vision_c1_AprilTag_Y_m>"
  Bus Selector20/3 -> Vision_Corrections/3  "<Vision_c1_AprilTag_Yaw_deg>"
  Bus Selector20/4 -> Vision_Corrections/4  "<Vision_c1_Object_Area_pct>"
  Bus Selector20/5 -> Vision_Corrections/5  "<Vision_c1_Object_Hor_deg>"
  Bus Selector20/6 -> Vision_Corrections/6  "<Vision_c1_Object_Ver_deg>"
  Human_Input_Pre_Processing/1 -> Bus Creator24/1
  Human_Input_Pre_Processing/2 -> Bus Creator24/2
  Unit Delay2/1 -> Human_Input_Pre_Processing/14  "Shooter_Active_prev"
  Bus Selector22/1 -> Unit Delay2/1  "<Shooter_Active>"
  Bus Selector1/7 -> Shooter Controls/7  "<Gamepad_RT>"
  Bus Selector13/6 -> Human_Input_Pre_Processing/6  "<Xbox_Driver_ButtonY>"
  Bus Selector13/7 -> Human_Input_Pre_Processing/7  "<Xbox_Driver_ButtonX>"
  Bus Selector13/8 -> Human_Input_Pre_Processing/8  "<Xbox_Driver_ButtonB>"
  Bus Selector13/13 -> Human_Input_Pre_Processing/13  "<Gyro_Angle_rad>"
  Shooter Controls/7 -> Bus Creator10/7
  Bus Selector7/4 -> Output Overrides/4(Desired_Shooter_Speed)  "<RB_Desired_Shooter_Speed>"
  Bus Selector7/5 -> Output Overrides/5(Desired_Shooter_FF_DC)  "<Desired_Shooter_FF_DC>"
  Bus Selector1/17 -> Shooter Controls/17  "<Gamepad_B2_B>"
  Shooter Controls/8 -> Bus Creator10/8
  Bus Selector23/1 -> Swerve_Drive/17  "<Aim_Active>"
  Shooter Controls/9 -> Bus Creator10/9
  Shooter Controls/10 -> Bus Creator10/10
  Shooter Controls/11 -> Bus Creator10/11
  Bus Selector24/1 -> Shooter_Motor_Gain_Kp/1  "<Shooter_Motor_Gain_Kp>"
  Bus Selector24/2 -> Shooter_Motor_Gain_Ki/1  "<Shooter_Motor_Gain_Ki>"
  Bus Selector24/3 -> Shooter_Motor_Gain_Change/1  "<Shooter_Motor_Gain_Change>"
  Bus Selector25/1 -> Intake Controls/7  "<RB_Transfer_Motor_PID_DC>"
  Teleop/8 -> Bus Creator2/8
  Teleop/9 -> Bus Creator2/9
  Teleop/10 -> Bus Creator2/10
  Teleop/11 -> Bus Creator2/11
  Teleop/12 -> Bus Creator2/12
  Teleop/13 -> Bus Creator2/13
  Teleop/14 -> Bus Creator2/14
  Teleop/15 -> Bus Creator2/15
  Teleop/16 -> Bus Creator2/16
  Teleop/17 -> Bus Creator2/17
  Teleop/18 -> Bus Creator2/18
  Teleop/19 -> Bus Creator2/19
  Teleop/20 -> Bus Creator2/20
  Teleop/21 -> Bus Creator2/21
  Teleop/22 -> Bus Creator2/22
  Autonomous/15 -> Bus Creator1/15
  Autonomous/16 -> Bus Creator1/16
  Autonomous/17 -> Bus Creator1/17
  Autonomous/18 -> Bus Creator1/18
  Autonomous/19 -> Bus Creator1/19
  Autonomous/20 -> Bus Creator1/20
  Autonomous/21 -> Bus Creator1/21
  Autonomous/22 -> Bus Creator1/22
  Disabled/15 -> Bus Creator4/15
  Disabled/16 -> Bus Creator4/16
  Disabled/17 -> Bus Creator4/17
  Disabled/18 -> Bus Creator4/18
  Disabled/19 -> Bus Creator4/19
  Disabled/20 -> Bus Creator4/20
  Disabled/21 -> Bus Creator4/21
  Disabled/22 -> Bus Creator4/22
  Test/15 -> Bus Creator12/15
  Test/16 -> Bus Creator12/16
  Test/17 -> Bus Creator12/17
  Test/18 -> Bus Creator12/18
  Test/19 -> Bus Creator12/19
  Test/20 -> Bus Creator12/20
  Test/21 -> Bus Creator12/21
  Test/22 -> Bus Creator12/22
  Bus Selector13/10 -> Human_Input_Pre_Processing/10  "<Gamepad_B3_X>"
  Bus Selector13/11 -> Human_Input_Pre_Processing/11  "<Gamepad_B4_Y>"
  Bus Selector13/12 -> Human_Input_Pre_Processing/12  "<Gamepad_B2_B>"
  Bus Selector1/18 -> Shooter Controls/18  "<Gamepad_Start>"
  Bus Selector13/9 -> Human_Input_Pre_Processing/9  "<Xbox_Driver_ButtonA>"
  Human_Input_Pre_Processing/3 -> Bus Creator24/3
  Human_Input_Pre_Processing/4 -> Bus Creator24/4
  Human_Input_Pre_Processing/5 -> Bus Creator24/5
  Human_Input_Pre_Processing/6 -> Bus Creator24/6
  Human_Input_Pre_Processing/7 -> Bus Creator24/7
  Human_Input_Pre_Processing/8 -> Bus Creator24/8
  Human_Input_Pre_Processing/9 -> Bus Creator24/9
  Human_Input_Pre_Processing/10 -> Bus Creator24/10
  Human_Input_Pre_Processing/11 -> Bus Creator24/11
  Human_Input_Pre_Processing/12 -> Bus Creator24/12
  Bus Selector41/3 -> Teleop/4  "<Steer_Joystick_X>"
  Bus Selector41/4 -> Teleop/5  "<Steer_Joystick_Y>"
  Bus Selector41/5 -> Teleop/6  "<Drive_Speed_Boost>"
  Bus Selector41/6 -> Teleop/7  "<Face_Toward_Driver>"
  Bus Selector41/7 -> Teleop/8  "<Face_Right_Driver>"
  Bus Selector41/8 -> Teleop/9  "<Face_Left_Driver>"
  Bus Selector41/9 -> Teleop/10  "<Face_Away_Driver>"
  Bus Selector41/10 -> Teleop/11  "<Gyro_Angle_rad>"
  Bus Selector41/11 -> Teleop/12  "<Prev_Active_GameState>"
  Bus Selector41/12 -> Teleop/13  "<IsBlueAlliance>"
  Bus Selector41/13 -> Teleop/14  "<Vision_Current_Pipeline>"
  Bus Selector41/14 -> Teleop/15  "<Vision_c1_AprilTag_Valid>"
  Bus Selector41/15 -> Teleop/16  "<Vision_c1_AprilTag_Corr_X_inch>"
  Bus Selector41/16 -> Teleop/17  "<Vision_c1_AprilTag_Corr_Y_inch>"
  Bus Selector41/17 -> Teleop/18  "<Vision_c1_AprilTag_Corr_Yaw_deg>"
  Bus Selector41/18 -> Teleop/19  "<Vision_c1_Object_Valid>"
  Bus Selector41/19 -> Teleop/20  "<Vision_c1_Object_Corr_X_inch>"
  Bus Selector41/20 -> Teleop/21  "<Vision_c1_Object_Corr_Y_inch>"
  Bus Selector41/21 -> Teleop/22  "<Vision_c1_Object_Corr_Yaw_deg>"
  Bus Selector41/22 -> Teleop/23  "<Gamepad_LB>"
  Bus Selector41/23 -> Teleop/24  "<Gamepad_RB>"
  Bus Selector41/24 -> Teleop/25  "<Gamepad_B1_A>"
  Bus Selector41/25 -> Teleop/26  "<Gamepad_B4_Y>"
  Bus Selector41/26 -> Teleop/27  "<Gamepad_B3_X>"
  Bus Selector41/27 -> Teleop/28  "<Xbox_Driver_Trigger_Left>"
  Bus Selector41/28 -> Teleop/29  "<Gamepad_LT>"

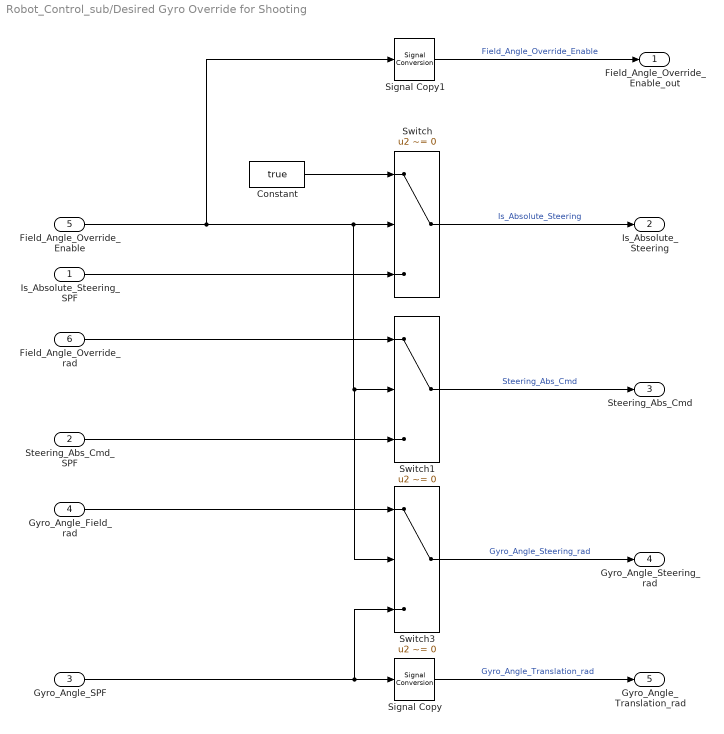
== system Robot_Control_sub/Desired Gyro Override for Shooting ==
  Is_Absolute_Steering_SPF : Inport
  Steering_Abs_Cmd_SPF : Inport  Port=2
  Gyro_Angle_SPF : Inport  Port=3
  Gyro_Angle_Field_rad : Inport  Port=4
  Field_Angle_Override_Enable : Inport  Port=5
  Field_Angle_Override_rad : Inport  Port=6
  Constant : Constant  Value=true
  Signal Copy : SignalConversion  OverrideOpt=off
  Signal Copy1 : SignalConversion  OverrideOpt=off
  Switch : Switch  Criteria=u2 ~= 0  SaturateOnIntegerOverflow=off  InputSameDT=off
  Switch1 : Switch  Criteria=u2 ~= 0  SaturateOnIntegerOverflow=off  InputSameDT=off
  Switch3 : Switch  Criteria=u2 ~= 0  SaturateOnIntegerOverflow=off  InputSameDT=off
  Field_Angle_Override_Enable_out : Outport
  Is_Absolute_Steering : Outport  Port=2
  Steering_Abs_Cmd : Outport  Port=3
  Gyro_Angle_Steering_rad : Outport  Port=4
  Gyro_Angle_Translation_rad : Outport  Port=5
  wires:
  Signal Copy1/1 -> Field_Angle_Override_Enable_out/1  "Field_Angle_Override_Enable"
  Signal Copy/1 -> Gyro_Angle_Translation_rad/1  "Gyro_Angle_Translation_rad"
  Gyro_Angle_Field_rad/1 -> Switch3/1
  Switch3/1 -> Gyro_Angle_Steering_rad/1  "Gyro_Angle_Steering_rad"
  Constant/1 -> Switch/1
  Switch1/1 -> Steering_Abs_Cmd/1  "Steering_Abs_Cmd"
  Switch/1 -> Is_Absolute_Steering/1  "Is_Absolute_Steering"
  Field_Angle_Override_rad/1 -> Switch1/1
  Gyro_Angle_SPF/1 -> Signal Copy/1, Switch3/3
  Steering_Abs_Cmd_SPF/1 -> Switch1/3
  Is_Absolute_Steering_SPF/1 -> Switch/3
  Field_Angle_Override_Enable/1 -> Switch/2, Switch1/2, Switch3/2, Signal Copy1/1

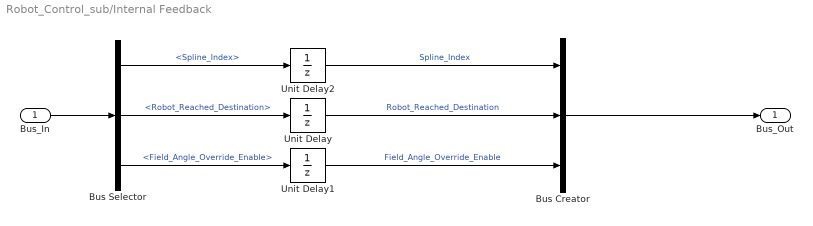
== system Robot_Control_sub/Internal Feedback ==
  Bus_In : Inport
  Bus Creator : BusCreator  Inputs=3
  Bus Selector : BusSelector  OutputSignals=SPF.Spline_Index,SPF.Robot_Reached_Destination,Desired_Gyro_Override.Field_Angle_Override_Enable
  Unit Delay : UnitDelay  SampleTime=-1
  Unit Delay1 : UnitDelay  SampleTime=-1
  Unit Delay2 : UnitDelay  InitialCondition=1  SampleTime=-1
  Bus_Out : Outport
  wires:
  Unit Delay2/1 -> Bus Creator/1  "Spline_Index"
  Bus Selector/1 -> Unit Delay2/1  "<Spline_Index>"
  Bus Creator/1 -> Bus_Out/1
  Unit Delay1/1 -> Bus Creator/3  "Field_Angle_Override_Enable"
  Bus Selector/3 -> Unit Delay1/1  "<Field_Angle_Override_Enable>"
  Unit Delay/1 -> Bus Creator/2  "Robot_Reached_Destination"
  Bus Selector/2 -> Unit Delay/1  "<Robot_Reached_Destination>"
  Bus_In/1 -> Bus Selector/1
